simulink model "simulink2_non_inverted_pend_ss_model_w_friction"  (R2026b)
settings: Solver=VariableStepAuto  StopTime=20.0
values from neighbouring files (symbols this model uses):
  A = [0 0 1 0 ... (first row only)    [setup_non_inverted_pend_ss_model_w_friction.m]
  B = km * B / Rm    [setup_non_inverted_pend_ss_model_w_friction.m]
  C = eye(2,4)    [setup_non_inverted_pend_ss_model_w_friction.m]
  D = zeros(2,1)    [setup_non_inverted_pend_ss_model_w_friction.m]
settings Model: Creator=leelou  LastModifiedBy=leelou

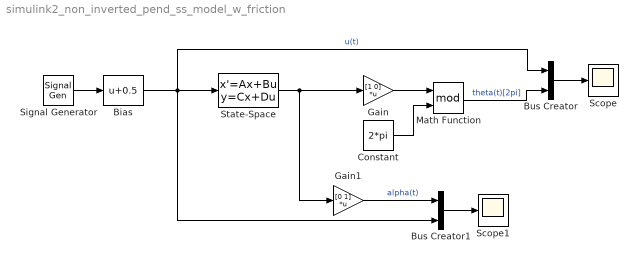
== system simulink2_non_inverted_pend_ss_model_w_friction ==
  Bias : Bias  Bias=0.5  SaturateOnIntegerOverflow=off
  Bus Creator : BusCreator  Inputs=2
  Bus Creator1 : BusCreator  Inputs=2
  Constant : Constant  Value=2*pi
  Gain : Gain  Gain=[1 0]  Multiplication=Matrix(K*u) (u vector)
  Gain1 : Gain  Gain=[0 1]  Multiplication=Matrix(K*u) (u vector)
  Math Function : Math  Operator=mod
  Scope : Scope
      settings: ActiveDisplayYMinimum=-0.12499999999999997  ActiveDisplayYMaximum=1.125
  Scope1 : Scope
      settings: ActiveDisplayYMinimum=-0.12507375876327187  ActiveDisplayYMaximum=1.1250081954181412
  Signal Generator : SignalGenerator  WaveForm=square  Amplitude=0.5
  State-Space : StateSpace  A=A  B=B  C=C  D=D  InitialCondition=0
  wires:
  Bus Creator/1 -> Scope/1
  Signal Generator/1 -> Bias/1
  Bias/1 -> Bus Creator1/2, State-Space/1, Bus Creator/1  "u(t)"
  State-Space/1 -> Gain1/1, Gain/1
  Bus Creator1/1 -> Scope1/1
  Gain1/1 -> Bus Creator1/1  "alpha(t)"
  Gain/1 -> Math Function/1
  Constant/1 -> Math Function/2
  Math Function/1 -> Bus Creator/2  "theta(t)[2pi]"
